simulink model "kalman_manuel_sim"  (R2026b)
settings: Solver=VariableStepAuto  StopTime=1500
values from neighbouring files (symbols this model uses):
  A = [ ... (first row only)    [model.m]
  Ad = sysd.A    [kalman_manuel.m]    (also in kalman_simulink.m)
  B = [1 / Cth_Res; 0; 0; 0; 0]    [model.m]
  Bd = sysd.B    [kalman_manuel.m]    (also in kalman_simulink.m = sysd.B(:, 1))
  C = eye(5)    [model.m]
  C_meas = [1 0 0 0 0 ... (first row only)    [kalman_manuel.m]    (also in kalman_simulink.m)
  E = [0; 0; (1 / Rv + 1 / R_pet) / Cth_air; 0; 0]    [model.m]
  Q = 1e-3 * eye(5)    [kalman_manuel.m]    (also in kalman_simulink.m)
  R = [0.245637158512  0; 0  0.335511625509]    [R_from_logs.mat]    (also in estimate_R.m = R_diag; kalman_manuel.m = diag([0.4956^2, 0.5792^2]); kalman_simulink.m = diag([0.4956^2, 0.5792^2]))
  Ts = 1    [R_from_logs.mat]    (also in estimate_R.m; kalman_manuel.m; kalman_simulink.m; model_file.m)
  x_IC = Tamb * ones(5, 1)    [kalman_manuel.m]
undefined symbols (not defined in the file or in its folder): DiscIntNeverNeededParam
settings Model: Creator=nael  LastModifiedBy=nael
settings DataIOCC: ExternalInput=data_in  LoadExternalInput=on
settings RTWCC: GPUComputeCapability=5.0

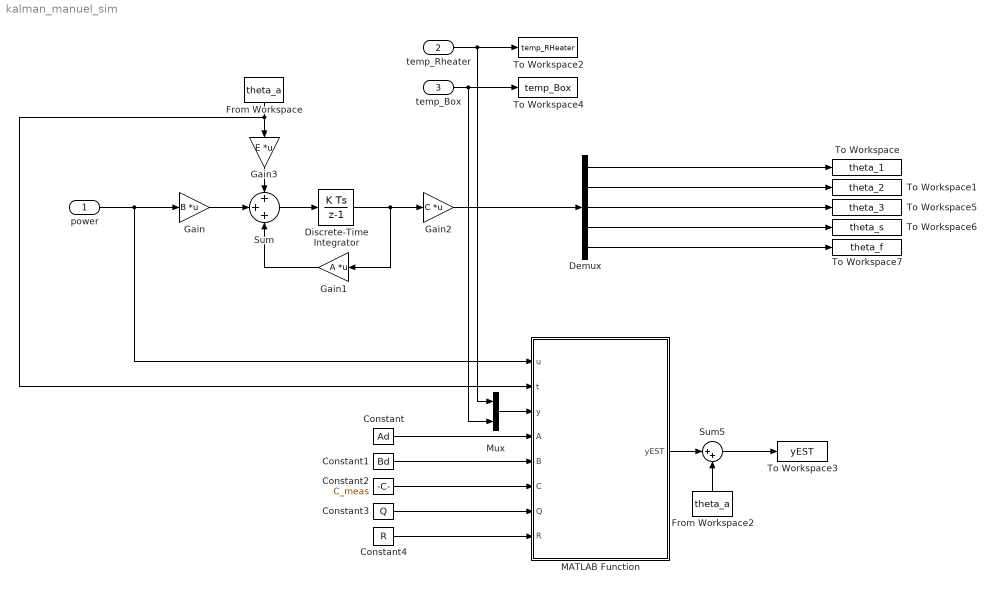
== system kalman_manuel_sim ==
  power : Inport
  temp_Rheater : Inport  Port=2
  temp_Box : Inport  Port=3
  Constant : Constant  Value=Ad  SampleTime=Ts
  Constant1 : Constant  Value=Bd  SampleTime=Ts
  Constant2 : Constant  Value=C_meas  VectorParams1D=off  SampleTime=Ts
  Constant3 : Constant  Value=Q  SampleTime=Ts
  Constant4 : Constant  Value=R  VectorParams1D=off  SampleTime=Ts
  Demux : Demux  Outputs=5
  Discrete-Time Integrator : DiscreteIntegrator  InitialCondition=x_IC  SampleTime=Ts  ICPrevOutput=DiscIntNeverNeededParam  ICPrevScaledInput=DiscIntNeverNeededParam
  From Workspace : FromWorkspace  VariableName=theta_a  SampleTime=Ts
  From Workspace2 : FromWorkspace  VariableName=theta_a  SampleTime=Ts
  Gain : Gain  Gain=B  Multiplication=Matrix(K*u)
  Gain1 : Gain  Gain=A  Multiplication=Matrix(K*u)
  Gain2 : Gain  Gain=C  Multiplication=Matrix(K*u)
  Gain3 : Gain  Gain=E  Multiplication=Matrix(K*u)
  MATLAB Function : MATLAB Function  TreatAsAtomicUnit=on  SystemSampleTime=Ts
  Mux : Mux  Inputs=2
  Sum : Sum  Inputs=+++
  Sum5 : Sum  Inputs=|++
  To Workspace : ToWorkspace  VariableName=theta_1  SampleTime=Ts
  To Workspace1 : ToWorkspace  VariableName=theta_2  SampleTime=Ts
  To Workspace2 : ToWorkspace  VariableName=temp_RHeater  SampleTime=Ts
  To Workspace3 : ToWorkspace  VariableName=yEST  SampleTime=Ts
      settings: Save2DSignal=2-D array (concatenate along first dimension)
  To Workspace4 : ToWorkspace  VariableName=temp_Box  SampleTime=Ts
  To Workspace5 : ToWorkspace  VariableName=theta_3  SampleTime=Ts
  To Workspace6 : ToWorkspace  VariableName=theta_s  SampleTime=Ts
  To Workspace7 : ToWorkspace  VariableName=theta_f  SampleTime=Ts
  wires:
  Gain1/1 -> Sum/3
  temp_Box/1 -> To Workspace4/1, Mux/2
  temp_Rheater/1 -> To Workspace2/1, Mux/1
  Demux/4 -> To Workspace6/1
  power/1 -> Gain/1, MATLAB Function/1(u)
  Demux/1 -> To Workspace/1
  Demux/3 -> To Workspace5/1
  Demux/5 -> To Workspace7/1
  Gain2/1 -> Demux/1
  MATLAB Function/1(yEST) -> Sum5/1
  Demux/2 -> To Workspace1/1
  Sum5/1 -> To Workspace3/1
  Gain/1 -> Sum/2
  From Workspace2/1 -> Sum5/2
  From Workspace/1 -> Gain3/1, MATLAB Function/2(t)
  Constant3/1 -> MATLAB Function/7(Q)
  Sum/1 -> Discrete-Time Integrator/1
  Constant4/1 -> MATLAB Function/8(R)
  Discrete-Time Integrator/1 -> Gain1/1, Gain2/1
  Gain3/1 -> Sum/1
  Constant2/1 -> MATLAB Function/6(C)
  Constant1/1 -> MATLAB Function/5(B)
  Constant/1 -> MATLAB Function/4(A)
  Mux/1 -> MATLAB Function/3(y)

== matlab function kalman_manuel_sim/MATLAB Function ==
  data: u input double size=[1 1]; t input; yEST output double; y input; A input size=[5 5]; B input size=[5 1]; C input; Q input size=[5 5]; R input
function yEST = fcn(u,t,y,A,B,C,Q,R)

persistent xEST;
persistent P;

if isempty(P)
    P = 10*eye(5);
    xEST = [0 ; 0 ; 0 ; 0 ; 0];
end

% Predict Estimates
P = A*P*A' + Q;
% Compute Kalman Gain
K = (P*C') / (C*P*C' + R);
% Update Covariance Matrix
P = (eye(5)-K*C)*P*(eye(5)-K*C)' + K*R*K';

% Predict States (xEST)
xEST = A*xEST + B*u;
% Update States (en relatif par rapport à t = Tamb)
xEST = xEST + K*((y - t) - C*xEST);

yEST = C*xEST;
